simulink model "SMR_PrimaryDT_v1"  (R2022b)
settings: Solver=FixedStepAuto  StartTime=0.0  StopTime=3600 * 5  FixedStep=0.01  RelTol=1e-3
libraries: fl_lib x60, nesl_utility x30, SimscapeFluids_lib x8, ee_lib x2, simulink x1, slpidlib x1
(part 2 of 2)

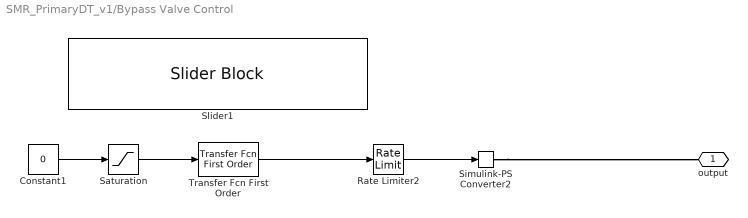
== system SMR_PrimaryDT_v1/Bypass Valve Control ==
  Constant1 : Constant  Value=0  OutMin=0  OutMax=1  OutDataTypeStr=double
  Rate Limiter2 : RateLimiter  RisingSlewLimit=0.02  FallingSlewLimit=-0.02  SampleTimeMode=inherited
  Saturation : Saturate  UpperLimit=1  LowerLimit=0
  Simulink-PS Converter2 : nesl_utility/Simulink-PS Converter  PhysicalDomain=network_engine_domain  SubClassName=ps_input  LeftPortType=input  RightPortType=output  PseudoPeriodic=off  Frequencies=[]  NoiseDistribution=none  NoiseParameters=[]  Unit=1  AffineConversion=off  FilteringAndDerivatives=provide  SimscapeFilterOrder=1  InputFilterTimeConstant=0.001  UdotUserProvided=0
  Slider1 : SliderBlock  ScaleMax=1  TickInterval=0.1
  Transfer Fcn First Order : simulink/Discrete/Transfer Fcn First Order  PoleZ=0.9802  ICPrevOutput=0.0  DoSatur=off
  output : PMIOPort  Side=Right
  wires:
  Constant1/1 -> Saturation/1
  Saturation/1 -> Transfer Fcn First Order/1
  Transfer Fcn First Order/1 -> Rate Limiter2/1
  Rate Limiter2/1 -> Simulink-PS Converter2/1
  connections:
  Simulink-PS Converter2/RConn1 -- output/RConn1

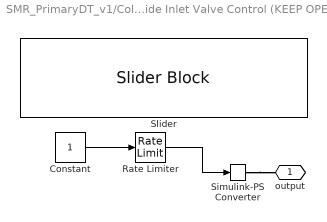
== system SMR_PrimaryDT_v1/Cold Side Inlet Valve Control (KEEP OPEN) ==
  Constant : Constant  OutMin=0  OutMax=1  OutDataTypeStr=double
  Rate Limiter : RateLimiter  RisingSlewLimit=0.1  FallingSlewLimit=-0.1  SampleTimeMode=inherited
  Simulink-PS Converter : nesl_utility/Simulink-PS Converter  PhysicalDomain=network_engine_domain  SubClassName=ps_input  LeftPortType=input  RightPortType=output  PseudoPeriodic=off  Frequencies=[]  NoiseDistribution=none  NoiseParameters=[]  Unit=1  AffineConversion=off  FilteringAndDerivatives=provide  SimscapeFilterOrder=1  InputFilterTimeConstant=0.001  UdotUserProvided=0
  Slider : SliderBlock  ScaleMin=0.02  ScaleMax=1  TickInterval=0.1
  output : PMIOPort  Side=Right
  wires:
  Constant/1 -> Rate Limiter/1
  Rate Limiter/1 -> Simulink-PS Converter/1
  connections:
  Simulink-PS Converter/RConn1 -- output/RConn1

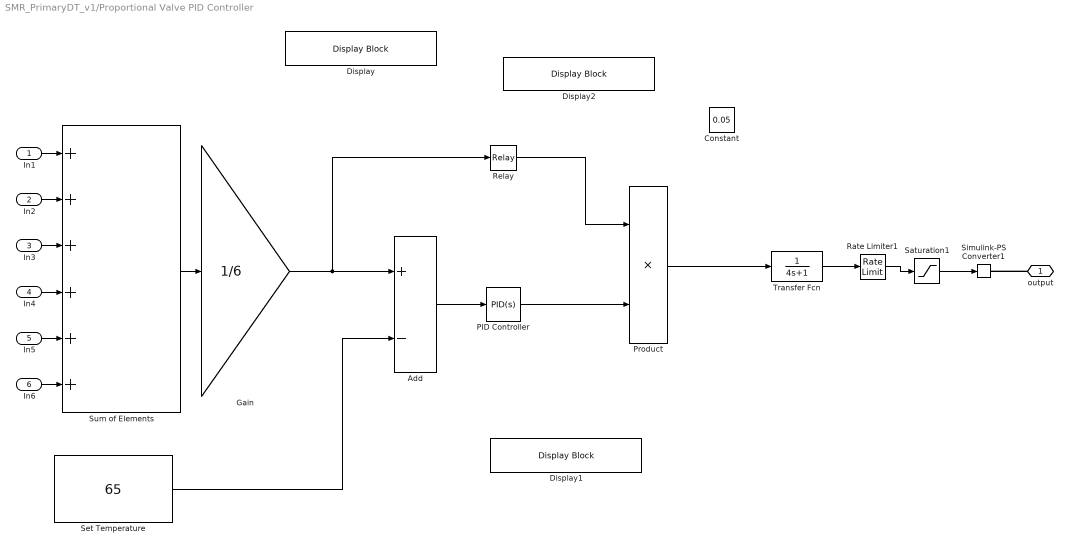
== system SMR_PrimaryDT_v1/Proportional Valve PID Controller ==
  In1 : Inport
  In2 : Inport  Port=2
  In3 : Inport  Port=3
  In4 : Inport  Port=4
  In5 : Inport  Port=5
  In6 : Inport  Port=6
  Add : Sum  Inputs=+-
  Constant : Constant  Value=0.05
  Display : DisplayBlock  LabelPosition=Hide  Transparency=1
  Display1 : DisplayBlock  LabelPosition=Hide  Transparency=1
  Display2 : DisplayBlock  LabelPosition=Hide  Transparency=1
  Gain : Gain  Gain=1/6
  PID Controller : slpidlib/PID Controller  Controller=PID  Form=Parallel  TimeDomain=Continuous-time  UseExternalTs=off  SampleTime=-1  IntegratorMethod=Forward Euler  FilterMethod=Forward Euler  ControllerParametersSource=internal  P=0.015  I=2e-5  UseKiTs=off  D=0  N=100  UseFilter=on  TunerSelectOption=Transfer Function Based (PID Tuner App)  InitialConditionSource=internal  InitialConditionForIntegrator=0  InitialConditionForFilter=0  DifferentiatorICPrevScaledInput=0  ExternalReset=none  TrackingMode=off  Kt=1  LimitOutput=on  SatLimitsSource=internal  UpperSaturationLimit=1  LowerSaturationLimit=0  LinearizeAsGain=on  AntiWindupMode=clamping  Kb=1  LimitIntegrator=off  UpperIntegratorSaturationLimit=inf  LowerIntegratorSaturationLimit=-inf  POutMin=[]  POutMax=[]  IOutMin=[]  IOutMax=[]  DOutMin=[]  DOutMax=[]  NOutMin=[]  NOutMax=[]  SumOutMin=[]  SumOutMax=[]  SaturationOutMin=[]  SaturationOutMax=[]  PParamMin=[]  PParamMax=[]  IParamMin=[]  IParamMax=[]  DParamMin=[]  DParamMax=[]  NParamMin=[]  NParamMax=[]  KbParamMin=[]  KbParamMax=[]  KtParamMin=[]  KtParamMax=[]  KbOutMin=[]  KbOutMax=[]  KtOutMin=[]  KtOutMax=[]  IntegratorOutMin=[]  IntegratorOutMax=[]  FilterOutMin=[]  FilterOutMax=[]  SumI1OutMin=[]  SumI1OutMax=[]  SumI2OutMin=[]  SumI2OutMax=[]  SumI3OutMin=[]  SumI3OutMax=[]  SumI4OutMin=[]  SumI4OutMax=[]  SumDOutMin=[]  SumDOutMax=[]  DifferentiatorOutMin=[]  DifferentiatorOutMax=[]  FilterDiffOutCoefMin=[]  FilterDiffOutCoefMax=[]  ReciprocalOutMin=[]  ReciprocalOutMax=[]  SumDenOutMin=[]  SumDenOutMax=[]  SumNumOutMin=[]  SumNumOutMax=[]  DivideOutMin=[]  DivideOutMax=[]  UdiffTsProdOutMin=[]  UdiffTsProdOutMax=[]  NTsProdOutMin=[]  NTsProdOutMax=[]  UintegralTsProdOutMin=[]  UintegralTsProdOutMax=[]  UngainTsProdOutMin=[]  UngainTsProdOutMax=[]  ClampingZeroOutDataTypeStr=Inherit: Inherit via back propagation  ClampingZeroOutMin=[]  ClampingZeroOutMax=[]  FilterDenConstantOutDataTypeStr=Inherit: Inherit via back propagation  FilterDenConstantOutMin=[]  FilterDenConstantOutMax=[]  PCopyOutDataTypeStr=Inherit: Inherit via back propagation  PCopyOutMin=[]  PCopyOutMax=[]  NCopyOutDataTypeStr=Inherit: Inherit via back propagation  NCopyOutMin=[]  NCopyOutMax=[]  IntegratorContinuousStateAttributes=''  IntegratorStateMustResolveToSignalObject=off  IntegratorRTWStateStorageClass=Auto  FilterContinuousStateAttributes=''  FilterStateMustResolveToSignalObject=off  FilterRTWStateStorageClass=Auto  ParallelPVariant=InternalParameters  IdealPVariant=Disabled  IVariant=InternalParameters  DVariant=InternalParameters  IntegratorVariant=Continuous  SatVariant=Enabled  AWVariant=ContClampingParallel  PCopyVariant=Disabled  TRVariant=Disabled  FdbkBlocksVariant=Forward  IdealPFdbkVariant=Disabled  SatFdbkVariant=Disabled  DerivativeFilterVariant=ContFilter  NVariant=InternalParameters  NCopyVariant=Disabled  FilterICVariant=InternalICsFilter  IntegratorICVariant=InternalICs  ExternalResetVariant=Disabled  TRSumVariant=Passthrough  SumFdbkVariant=Disabled  SumVariant=Sum_PID  TsampFilterVariant=InternalTs  TsampNgainVariant=Passthrough  TsampIntegralVariant=Passthrough  ExternalSaturationOutDataTypeStr=Inherit: Same as second input
  Product : Product
  Rate Limiter1 : RateLimiter  RisingSlewLimit=0.03  FallingSlewLimit=-0.08  SampleTimeMode=inherited  LinearizeAsGain=off
  Relay : Relay  OnSwitchValue=63  OffSwitchValue=62
  Saturation1 : Saturate  UpperLimit=1  LowerLimit=0
  Set Temperature : Constant  Value=65
  Simulink-PS Converter1 : nesl_utility/Simulink-PS Converter  PhysicalDomain=network_engine_domain  SubClassName=ps_input  LeftPortType=input  RightPortType=output  PseudoPeriodic=off  Frequencies=[]  NoiseDistribution=none  NoiseParameters=[]  Unit=1  AffineConversion=off  FilteringAndDerivatives=provide  SimscapeFilterOrder=1  InputFilterTimeConstant=0.001  UdotUserProvided=0
  Sum of Elements : Sum  Inputs=++++++
  Transfer Fcn : TransferFcn  Denominator=[4 1]
  output : PMIOPort  Side=Right
  wires:
  Sum of Elements/1 -> Gain/1
  Rate Limiter1/1 -> Saturation1/1
  Set Temperature/1 -> Add/2
  In1/1 -> Sum of Elements/1
  In2/1 -> Sum of Elements/2
  In3/1 -> Sum of Elements/3
  In4/1 -> Sum of Elements/4
  In5/1 -> Sum of Elements/5
  In6/1 -> Sum of Elements/6
  Product/1 -> Transfer Fcn/1
  Transfer Fcn/1 -> Rate Limiter1/1
  Saturation1/1 -> Simulink-PS Converter1/1
  Gain/1 -> Relay/1, Add/1
  Add/1 -> PID Controller/1
  PID Controller/1 -> Product/2
  Relay/1 -> Product/1
  connections:
  output/RConn1 -- Simulink-PS Converter1/RConn1
